simulink model "hybrid_pv_wind_feeder"  (R2024b)
settings: Solver=FixedStepDiscrete  StartTime=0.0  StopTime=1.0  FixedStep=P.Ts  RelTol=1e-3
model workspace (MAT data in the model file):
  P : object (value not decoded)
symbols that are objects in the model workspace (value not decoded): P
undefined symbols (not defined in the file): DiscIntNeverNeededParam
libraries: spsThreePhaseSeriesRLCBranchLib x28, spsSeriesRLCBranchLib x14, spsThreePhaseParallelRLCLoadLib x12, spsIGBTDiodeLib x8, slpidlib x7, spsThreePhaseBreakerLib x6, simulink x4, spsGroundLib x4, spsThreePhaseVIMeasurementLib x4, spsControlledCurrentSourceLib x3, spsDiodeLib x2, spsAlphaBetaZerotodq0Lib x2
(part 2 of 2)

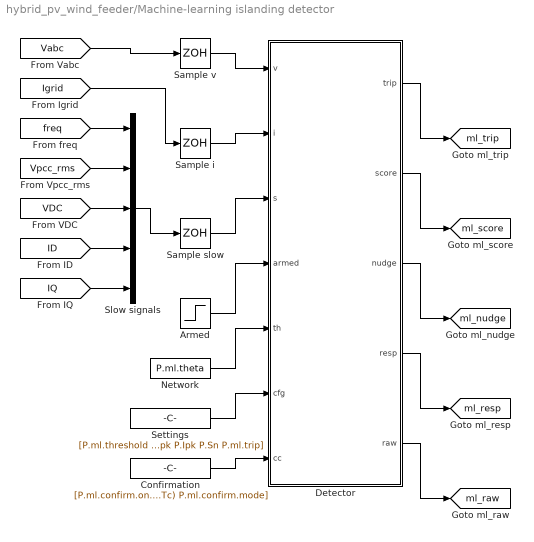
== system hybrid_pv_wind_feeder/Machine-learning islanding detector ==
  Armed : Step  Time=P.ml.tArm  SampleTime=P.Tc
  Confirmation : Constant  Value=[P.ml.confirm.on P.ml.confirm.amp round(P.ml.confirm.T/P.Tc) P.ml.confirm.thr P.ml.confirm.sign round(P.ml.confirm.hold/P.Tc) P.ml.confirm.mode]
  Detector : MATLAB Function  TreatAsAtomicUnit=on
  Network : Constant  Value=P.ml.theta
  Sample i : ZeroOrderHold  SampleTime=P.Tc
  Sample slow : ZeroOrderHold  SampleTime=P.Tc
  Sample v : ZeroOrderHold  SampleTime=P.Tc
  Settings : Constant  Value=[P.ml.threshold P.ml.debounce P.Vpk P.Ipk P.Sn P.ml.trip]
  Slow signals : Mux  Inputs=5
  tag scope: ml_nudge=global, ml_raw=global, ml_resp=global, ml_score=global, ml_trip=global
  wires:
  [freq] -> Slow signals/1
  [Vpcc_rms] -> Slow signals/2
  [VDC] -> Slow signals/3
  [ID] -> Slow signals/4
  [IQ] -> Slow signals/5
  [Vabc] -> Sample v/1
  [Igrid] -> Sample i/1
  Slow signals/1 -> Sample slow/1
  Sample v/1 -> Detector/1(v)
  Sample i/1 -> Detector/2(i)
  Sample slow/1 -> Detector/3(s)
  Armed/1 -> Detector/4(armed)
  Network/1 -> Detector/5(th)
  Settings/1 -> Detector/6(cfg)
  Confirmation/1 -> Detector/7(cc)
  Detector/1(trip) -> [ml_trip]
  Detector/2(score) -> [ml_score]
  Detector/3(nudge) -> [ml_nudge]
  Detector/4(resp) -> [ml_resp]
  Detector/5(raw) -> [ml_raw]

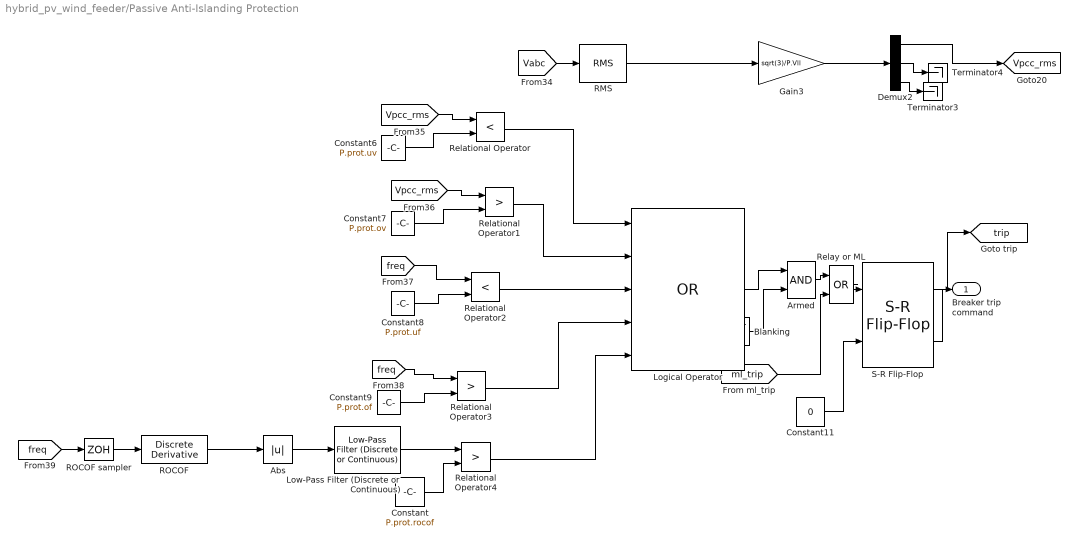
== system hybrid_pv_wind_feeder/Passive Anti-Islanding Protection ==
  Abs : Abs  SaturateOnIntegerOverflow=off
  Armed : Logic  AllPortsSameDT=off  OutDataTypeStr=boolean
  Blanking : Step  Time=P.prot.tArm  SampleTime=P.Ts
  Constant : Constant  Value=P.prot.rocof
  Constant11 : Constant  Value=0  VectorParams1D=off  OutDataTypeStr=boolean
  Constant6 : Constant  Value=P.prot.uv
  Constant7 : Constant  Value=P.prot.ov
  Constant8 : Constant  Value=P.prot.uf
  Constant9 : Constant  Value=P.prot.of
  Demux2 : Demux  Outputs=3
  Gain3 : Gain  Gain=sqrt(3)/P.Vll
  Logical Operator : Logic  Operator=OR  Inputs=5  AllPortsSameDT=off  OutDataTypeStr=boolean
  Low-Pass Filter (Discrete or Continuous) : eeGeneralControl/Low-Pass Filter (Discrete or Continuous)  K=1  T=1/(2*pi*10)  B=inf  A=-inf  init_option=Inherited from block input  x0=0  Ts=-1
  RMS : spsRMSLib/RMS  TrueRMS=on  Freq=P.fg  RMSInit=120  Ts=P.Ts
  ROCOF : simulink/Discrete/Discrete Derivative  gainval=1.0  ICPrevScaledInput=0.0  OutMin=[]  OutMax=[]  OutDataType=fixdt(1, 16)  OutScaling=2^-10  DoSatur=off
  ROCOF sampler : ZeroOrderHold  SampleTime=P.prot.Trocof
  Relational Operator : RelationalOperator  Operator=<  OutDataTypeStr=boolean  RndMeth=Simplest  InputSameDT=off
  Relational Operator1 : RelationalOperator  Operator=>  OutDataTypeStr=boolean  RndMeth=Simplest  InputSameDT=off
  Relational Operator2 : RelationalOperator  Operator=<  OutDataTypeStr=boolean  RndMeth=Simplest  InputSameDT=off
  Relational Operator3 : RelationalOperator  Operator=>  OutDataTypeStr=boolean  RndMeth=Simplest  InputSameDT=off
  Relational Operator4 : RelationalOperator  Operator=>  OutDataTypeStr=boolean  RndMeth=Simplest  InputSameDT=off
  Relay or ML : Logic  Operator=OR  AllPortsSameDT=off  OutDataTypeStr=boolean
  S-R Flip-Flop : simulink_extras/Flip Flops/S-R Flip-Flop  initial_condition=0
  Terminator3 : Terminator
  Terminator4 : Terminator
  "Breaker trip command " : Outport  VectorParamsAs1DForOutWhenUnconnected=off
  tag scope: Vpcc_rms=global, trip=global
  wires:
  RMS/1 -> Gain3/1
  Constant6/1 -> Relational Operator/2
  Constant7/1 -> Relational Operator1/2
  Abs/1 -> Low-Pass Filter (Discrete or Continuous)/1
  [Vpcc_rms] -> Relational Operator1/1
  Gain3/1 -> Demux2/1
  [Vabc] -> RMS/1
  [freq] -> Relational Operator3/1
  Low-Pass Filter (Discrete or Continuous)/1 -> Relational Operator4/1
  Constant11/1 -> S-R Flip-Flop/2
  Demux2/1 -> [Vpcc_rms]
  Constant8/1 -> Relational Operator2/2
  Constant/1 -> Relational Operator4/2
  Constant9/1 -> Relational Operator3/2
  [Vpcc_rms] -> Relational Operator/1
  Demux2/2 -> Terminator4/1
  Relational Operator1/1 -> Logical Operator/2
  Demux2/3 -> Terminator3/1
  Relational Operator3/1 -> Logical Operator/4
  Relational Operator/1 -> Logical Operator/1
  Relational Operator2/1 -> Logical Operator/3
  [freq] -> Relational Operator2/1
  Relational Operator4/1 -> Logical Operator/5
  [freq] -> ROCOF sampler/1
  ROCOF sampler/1 -> ROCOF/1
  ROCOF/1 -> Abs/1
  Logical Operator/1 -> Armed/1
  Blanking/1 -> Armed/2
  Armed/1 -> Relay or ML/1
  [ml_trip] -> Relay or ML/2
  Relay or ML/1 -> S-R Flip-Flop/1
  S-R Flip-Flop/2 -> "Breaker trip command "/1
  S-R Flip-Flop/1 -> [trip]

== system hybrid_pv_wind_feeder/Pwm Generator  ==
  1 : Inport
  Demux3 : Demux  Outputs=3
  Logical Operator1 : Logic  Operator=NOT  AllPortsSameDT=off  OutDataTypeStr=boolean
  Logical Operator2 : Logic  Operator=NOT  AllPortsSameDT=off  OutDataTypeStr=boolean
  Logical Operator3 : Logic  Operator=NOT  AllPortsSameDT=off  OutDataTypeStr=boolean
  Relational Operator : RelationalOperator  OutDataTypeStr=boolean  RndMeth=Simplest  InputSameDT=off
  Relational Operator1 : RelationalOperator  OutDataTypeStr=boolean  RndMeth=Simplest  InputSameDT=off
  Relational Operator2 : RelationalOperator  OutDataTypeStr=boolean  RndMeth=Simplest  InputSameDT=off
  Repeating Sequence : simulink/Sources/Repeating Sequence  rep_seq_t=[0 0.00005 0.0001]  rep_seq_y=[-1 1 -1]
  tag scope: PWM1=global, PWM2=global, PWM3=global, PWM4=global, PWM5=global, PWM6=global
  wires:
  Relational Operator/1 -> Logical Operator1/1, [PWM1]
  Demux3/2 -> Relational Operator1/1
  Demux3/1 -> Relational Operator/1
  Relational Operator1/1 -> [PWM3], Logical Operator2/1
  Repeating Sequence/1 -> Relational Operator1/2, Relational Operator/2, Relational Operator2/2
  Demux3/3 -> Relational Operator2/1
  1/1 -> Demux3/1
  Relational Operator2/1 -> [PWM5], Logical Operator3/1
  Logical Operator1/1 -> [PWM2]
  Logical Operator2/1 -> [PWM4]
  Logical Operator3/1 -> [PWM6]

== system hybrid_pv_wind_feeder/Second inverter control ==
  Armed : Step  Time=P.prot.tBlank  SampleTime=P.der2.Ts
  Current reference : MATLAB Function  TreatAsAtomicUnit=on
  Delay : UnitDelay  SampleTime=P.der2.Ts  HasFrameUpgradeWarning=on
  Enable : Step  Time=P.der2.tOn  After=P.der2.on  SampleTime=P.der2.Ts
  Sample : ZeroOrderHold  SampleTime=P.der2.Ts
  Sample freq : ZeroOrderHold  SampleTime=P.der2.Ts
  Settings : Constant  Value=[P.der2.P P.der2.Q P.der2.Kq P.der2.Qlim P.fg 1.5*(0.5*P.Vll*sqrt(2/3))^2 P.der2.Ts]
  Iabc ref : Outport
  wires:
  [Vder2] -> Sample/1
  Sample/1 -> Current reference/1(v)
  Enable/1 -> Current reference/3(en)
  Armed/1 -> Current reference/4(armed)
  Settings/1 -> Current reference/5(prm)
  Current reference/1(i) -> Delay/1
  Delay/1 -> Iabc ref/1
  [freq] -> Sample freq/1
  Sample freq/1 -> Current reference/2(f)

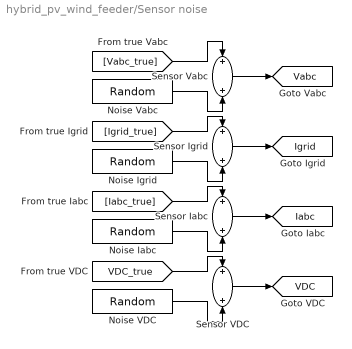
== system hybrid_pv_wind_feeder/Sensor noise ==
  Noise Iabc : RandomNumber  Variance=(P.noise.on*P.noise.i*P.Ipk)^2  Seed=10*P.noise.seed + [7 8 9]  SampleTime=P.Tc
  Noise Igrid : RandomNumber  Variance=(P.noise.on*P.noise.i*P.Ipk)^2  Seed=10*P.noise.seed + [4 5 6]  SampleTime=P.Tc
  Noise VDC : RandomNumber  Variance=(P.noise.on*P.noise.vdc*P.Vdc)^2  Seed=10*P.noise.seed + 10  SampleTime=P.Tc
  Noise Vabc : RandomNumber  Variance=(P.noise.on*P.noise.v*P.Vpk)^2  Seed=10*P.noise.seed + [1 2 3]  SampleTime=P.Tc
  Sensor Iabc : Sum
  Sensor Igrid : Sum
  Sensor VDC : Sum
  Sensor Vabc : Sum
  tag scope: Iabc=global, Igrid=global, VDC=global, Vabc=global
  wires:
  [Vabc_true] -> Sensor Vabc/1
  Noise Vabc/1 -> Sensor Vabc/2
  Sensor Vabc/1 -> [Vabc]
  [Igrid_true] -> Sensor Igrid/1
  Noise Igrid/1 -> Sensor Igrid/2
  Sensor Igrid/1 -> [Igrid]
  [Iabc_true] -> Sensor Iabc/1
  Noise Iabc/1 -> Sensor Iabc/2
  Sensor Iabc/1 -> [Iabc]
  [VDC_true] -> Sensor VDC/1
  Noise VDC/1 -> Sensor VDC/2
  Sensor VDC/1 -> [VDC]

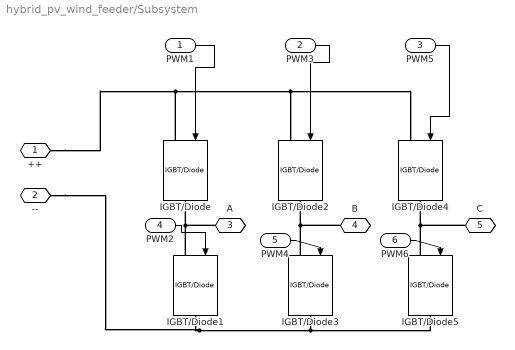
== system hybrid_pv_wind_feeder/Subsystem ==
  PWM1 : Inport
  PWM3 : Inport  Port=2
  PWM5 : Inport  Port=3
  PWM2 : Inport  Port=4
  PWM4 : Inport  Port=5
  PWM6 : Inport  Port=6
  IGBT/Diode{,1..5} (6 alike) : spsIGBTDiodeLib/IGBT//Diode  Ron=1e-3  Rs=1e5  Cs=inf  Measurements=off
  ++ : PMIOPort  Side=Left
  -- : PMIOPort  Port=2  Side=Left
  A : PMIOPort  Port=3  Side=Right
  B : PMIOPort  Port=4  Side=Right
  C : PMIOPort  Port=5  Side=Right
  wires:
  PWM1/1 -> IGBT/Diode/1
  PWM4/1 -> IGBT/Diode3/1
  PWM6/1 -> IGBT/Diode5/1
  PWM3/1 -> IGBT/Diode2/1
  PWM5/1 -> IGBT/Diode4/1
  PWM2/1 -> IGBT/Diode1/1
  connections:
  IGBT/Diode1/RConn1 -- --/RConn1 -- IGBT/Diode3/RConn1 -- IGBT/Diode5/RConn1
  IGBT/Diode3/LConn1 -- B/RConn1 -- IGBT/Diode2/RConn1
  IGBT/Diode1/LConn1 -- A/RConn1 -- IGBT/Diode/RConn1
  IGBT/Diode5/LConn1 -- C/RConn1 -- IGBT/Diode4/RConn1
  IGBT/Diode/LConn1 -- ++/RConn1 -- IGBT/Diode2/LConn1 -- IGBT/Diode4/LConn1

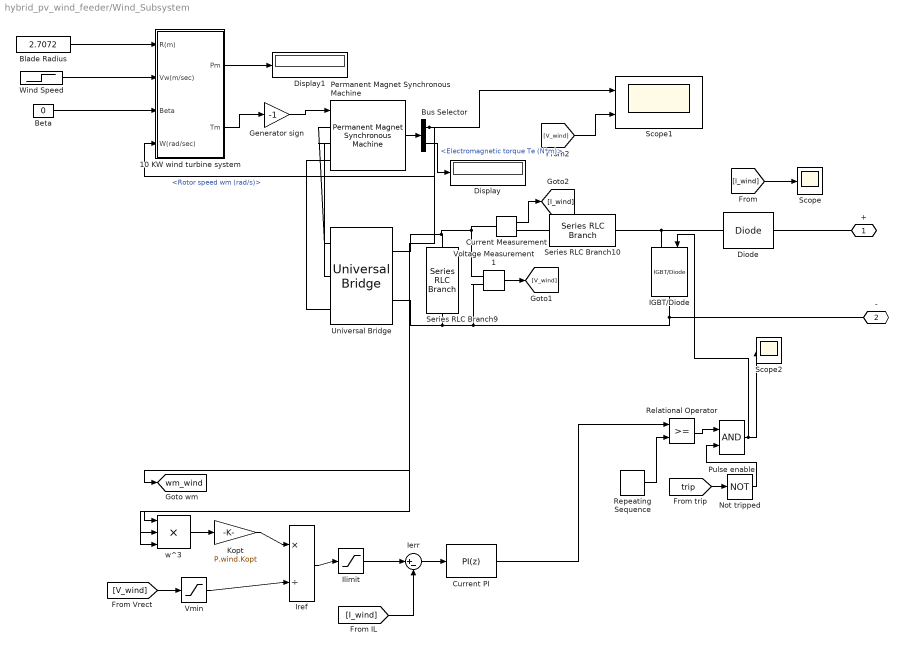
== system hybrid_pv_wind_feeder/Wind_Subsystem ==
  10 KW wind turbine system : Subsystem
  Beta : Constant  Value=0
  Blade Radius : Constant  Value=2.7072
  Bus Selector : BusSelector  OutputSignals=Rotor speed wm (rad/s),Electromagnetic torque Te (N*m)
  Current Measurement : spsCurrentMeasurementLib/Current Measurement  PhasorSimulation=off  OutputType=Complex  PSBequivalent=0
  Current PI : slpidlib/PID Controller  Controller=PI  Form=Parallel  TimeDomain=Discrete-time  UseExternalTs=off  SampleTime=-1  IntegratorMethod=Forward Euler  FilterMethod=Forward Euler  ControllerParametersSource=internal  P=P.wind.KpI  I=P.wind.KiI  UseKiTs=off  D=0  UseExternalDerivativeSource=off  N=100  UseFilter=on  TunerSelectOption=Transfer Function Based (PID Tuner App)  InitialConditionSource=internal  InitialConditionForIntegrator=P.wind.D0  InitialConditionForFilter=0  DifferentiatorICPrevScaledInput=0  ExternalReset=none  TrackingMode=off  Kt=1  LimitOutput=on  SatLimitsSource=internal  UpperSaturationLimit=0.92  LowerSaturationLimit=0  LinearizeAsGain=off  AntiWindupMode=clamping  Kb=1  LimitIntegrator=off  UpperIntegratorSaturationLimit=inf  LowerIntegratorSaturationLimit=-inf  POutMin=[]  POutMax=[]  IOutMin=[]  IOutMax=[]  DOutMin=[]  DOutMax=[]  NOutMin=[]  NOutMax=[]  SumOutMin=[]  SumOutMax=[]  SaturationOutMin=[]  SaturationOutMax=[]  PParamMin=[]  PParamMax=[]  IParamMin=[]  IParamMax=[]  DParamMin=[]  DParamMax=[]  NParamMin=[]  NParamMax=[]  KbParamMin=[]  KbParamMax=[]  KtParamMin=[]  KtParamMax=[]  KbOutMin=[]  KbOutMax=[]  KtOutMin=[]  KtOutMax=[]  IntegratorOutMin=[]  IntegratorOutMax=[]  FilterOutMin=[]  FilterOutMax=[]  SumI1OutMin=[]  SumI1OutMax=[]  SumI2OutMin=[]  SumI2OutMax=[]  SumI3OutMin=[]  SumI3OutMax=[]  SumI4OutMin=[]  SumI4OutMax=[]  SumDOutMin=[]  SumDOutMax=[]  DifferentiatorOutMin=[]  DifferentiatorOutMax=[]  FilterDiffOutCoefMin=[]  FilterDiffOutCoefMax=[]  ReciprocalOutMin=[]  ReciprocalOutMax=[]  SumDenOutMin=[]  SumDenOutMax=[]  SumNumOutMin=[]  SumNumOutMax=[]  DivideOutMin=[]  DivideOutMax=[]  UdiffTsProdOutMin=[]  UdiffTsProdOutMax=[]  NTsProdOutMin=[]  NTsProdOutMax=[]  UintegralTsProdOutMin=[]  UintegralTsProdOutMax=[]  UngainTsProdOutMin=[]  UngainTsProdOutMax=[]  ClampingZeroOutDataTypeStr=Inherit: Inherit via back propagation  ClampingZeroOutMin=[]  ClampingZeroOutMax=[]  FilterDenConstantOutDataTypeStr=Inherit: Inherit via back propagation  FilterDenConstantOutMin=[]  FilterDenConstantOutMax=[]  PCopyOutDataTypeStr=Inherit: Inherit via back propagation  PCopyOutMin=[]  PCopyOutMax=[]  NCopyOutDataTypeStr=Inherit: Inherit via back propagation  NCopyOutMin=[]  NCopyOutMax=[]  IntegratorContinuousStateAttributes=''  IntegratorStateMustResolveToSignalObject=off  IntegratorRTWStateStorageClass=Auto  FilterContinuousStateAttributes=''  FilterStateMustResolveToSignalObject=off  FilterRTWStateStorageClass=Auto  ParallelPVariant=InternalParameters  IdealPVariant=Disabled  IVariant=InternalParameters  DVariant=Disabled  IntegratorVariant=Discrete  SatVariant=Enabled  AWVariant=DiscClampingParallel  PCopyVariant=Disabled  TRVariant=Disabled  FdbkBlocksVariant=Forward  IdealPFdbkVariant=Disabled  SatFdbkVariant=Disabled  DerivativeFilterVariant=Disabled  NVariant=Disabled  NCopyVariant=Disabled_SignalSpec  FilterICVariant=Disabled  IntegratorICVariant=InternalICs  ExternalResetVariant=Disabled  TRSumVariant=Passthrough  SumFdbkVariant=Disabled  SumVariant=Sum_PI  TsampFilterVariant=InternalTs  TsampNgainVariant=Passthrough  TsampIntegralVariant=Disabled_SignalSpec  ExternalSaturationOutDataTypeStr=Inherit: Same as second input  DerivativeSourceVariant=Disabled  PreIntVariant=InternalPreInt
      settings: LibrarySourceBlock=simulink/Discrete/Discrete PID Controller
  Diode : spsDiodeLib/Diode  Ron=0.001  Lon=0  Vf=0.8  IC=0  UseSnubber=0  Rs=500  Cs=250e-9  Measurements=off
  Display : Display
  Display1 : Display
  Generator sign : Gain  Gain=-1
  IGBT/Diode : spsIGBTDiodeLib/IGBT//Diode  Ron=0.001  Rs=100  Cs=1e-6  Measurements=off
  Ierr : Sum  Inputs=|+-
  Ilimit : Saturate  UpperLimit=P.wind.Imax  LowerLimit=0
  Iref : Product  Inputs=*/
  Kopt : Gain  Gain=P.wind.Kopt
  Not tripped : Logic  Operator=NOT  AllPortsSameDT=off  OutDataTypeStr=boolean
  Permanent Magnet Synchronous Machine : spsPermanentMagnetSynchronousMachineLib/Permanent Magnet Synchronous Machine  NbPhases=3  FluxDistribution=Sinusoidal  RotorType=Round  MechanicalLoad=Torque Tm  PresetModel=No  ShowDetailedParameters=on  MeasurementBus=off  Resistance=0.05486  Inductance=P.wind.Ls  dqInductances=[P.wind.Ls P.wind.Ls]  La=0.000835  MachineConstant=Flux linkage established by magnets (V.s)  Flux=0.9  VoltageCst=652.9678  TorqueCst=5.4  Flat=120  Mechanical=[P.wind.J 0.008 P.wind.pp 0]  PolePairs=P.wind.pp  InitialConditions=[P.wind.wm0 0 0 0]  InitialConditions5ph=[0 0 0 0 0 0]  RefAngle=90 degrees behind phase A axis (modified Park)  IterativeDiscreteModel=Trapezoidal non iterative  TsBlock=-1  TsPowergui=0
  Pulse enable : Logic  AllPortsSameDT=off  OutDataTypeStr=boolean
  Relational Operator : RelationalOperator  OutDataTypeStr=boolean  RndMeth=Simplest  InputSameDT=off
  Repeating Sequence : simulink/Sources/Repeating Sequence  rep_seq_t="[0  0.0001]"  rep_seq_y=[0 1]
  Scope : Scope
  Scope1 : Scope  NumInputPorts=2
  Scope2 : Scope
  Series RLC Branch10 : spsSeriesRLCBranchLib/Series RLC Branch  LConnTagsString=__new0  RConnTagsString=__new0  BranchType=L  Resistance=2.3e-3  Inductance=10e-3  SetiL0=off  InitialCurrent=0  Capacitance=1e-6  Setx0=off  InitialVoltage=0  Measurements=None
  Series RLC Branch9 : spsSeriesRLCBranchLib/Series RLC Branch  LConnTagsString=__new0  RConnTagsString=__new0  BranchType=C  Resistance=1  Inductance=1e-3  SetiL0=off  InitialCurrent=0  Capacitance=2200e-6  Setx0=off  InitialVoltage=0  Measurements=None
  Universal Bridge : spsUniversalBridgeLib/Universal Bridge  Arms=3  SnubberResistance=5000  SnubberCapacitance=inf  Device=Diodes  Ron=0.001  Lon=0  ForwardVoltages="[  0  0  ]"  ForwardVoltage=0  GTOparameters=[ 10e-6 , 20e-6 ]  IGBTparameters=[ 1e-6 , 2e-6 ]  Measurements=None  Measurements_2=None  converterType=Rectifier
  Vmin : Saturate  UpperLimit=inf  LowerLimit=50
  Voltage Measurement1 : spsVoltageMeasurementLib/Voltage Measurement  PhasorSimulation=off  OutputType=Complex  PSBequivalent=0
  Wind Speed : Step  Time=P.wind.tStep  Before=P.wind.v0  After=P.wind.v1  SampleTime=0
  w^3 : Product  Inputs=3
  + : PMIOPort  Side=Right
  - : PMIOPort  Port=2  Side=Right
  tag scope: wm_wind=global
  wires:
  Bus Selector/1 -> Scope1/1, 10 KW wind turbine system/4(W(rad/sec)), w^3/1, w^3/2, w^3/3, [wm_wind]  "<Rotor speed wm (rad/s)>"
  [V_wind] -> Scope1/2
  Repeating Sequence/1 -> Relational Operator/2
  Permanent Magnet Synchronous Machine/1 -> Bus Selector/1
  Bus Selector/2 -> Display/1  "<Electromagnetic torque Te (N*m)>"
  Voltage Measurement1/1 -> [V_wind]
  Current Measurement/1 -> [I_wind]
  Beta/1 -> 10 KW wind turbine system/3(Beta)
  Blade Radius/1 -> 10 KW wind turbine system/1(R(m))
  10 KW wind turbine system/1(Pm) -> Display1/1
  Wind Speed/1 -> 10 KW wind turbine system/2(Vw(m/sec))
  [I_wind] -> Scope/1
  10 KW wind turbine system/2(Tm) -> Generator sign/1
  Generator sign/1 -> Permanent Magnet Synchronous Machine/1
  w^3/1 -> Kopt/1
  Kopt/1 -> Iref/1
  [V_wind] -> Vmin/1
  Vmin/1 -> Iref/2
  Iref/1 -> Ilimit/1
  Ilimit/1 -> Ierr/1
  [I_wind] -> Ierr/2
  Ierr/1 -> Current PI/1
  Current PI/1 -> Relational Operator/1
  [trip] -> Not tripped/1
  Relational Operator/1 -> Pulse enable/1
  Not tripped/1 -> Pulse enable/2
  Pulse enable/1 -> Scope2/1, IGBT/Diode/1
  connections:
  Series RLC Branch9/LConn1 -- Universal Bridge/RConn1 -- Voltage Measurement1/LConn1 -- Current Measurement/LConn1
  IGBT/Diode/RConn1 -- Voltage Measurement1/LConn2 -- Universal Bridge/RConn2 -- Series RLC Branch9/RConn1 -- -/RConn1
  Series RLC Branch10/RConn1 -- Diode/LConn1 -- IGBT/Diode/LConn1
  Diode/RConn1 -- +/RConn1
  Permanent Magnet Synchronous Machine/LConn2 -- Universal Bridge/LConn2
  Permanent Magnet Synchronous Machine/LConn1 -- Universal Bridge/LConn1
  Current Measurement/RConn1 -- Series RLC Branch10/LConn1
  Permanent Magnet Synchronous Machine/LConn3 -- Universal Bridge/LConn3

== system hybrid_pv_wind_feeder/Inverter Control Logic/Active frequency drift ==
  Add bias : Sum
  Add nudge : Sum
  Armed : Step  Time=P.prot.tBlank  After=P.afd.on  SampleTime=P.Tc
  Enable : Product
  Frequency error : Sum  Inputs=+-
  K : Gain  Gain=P.afd.K
  Limit : Saturate  UpperLimit=P.afd.lim  LowerLimit=-P.afd.lim
  bias : Constant  Value=P.afd.bias
  fg : Constant  Value=P.fg
  Iq ref : Outport
  wires:
  [freq] -> Frequency error/1
  fg/1 -> Frequency error/2
  Frequency error/1 -> K/1
  K/1 -> Add bias/1
  bias/1 -> Add bias/2
  Add bias/1 -> Limit/1
  Limit/1 -> Enable/1
  Armed/1 -> Enable/2
  Enable/1 -> Add nudge/1
  [ml_nudge] -> Add nudge/2
  Add nudge/1 -> Iq ref/1

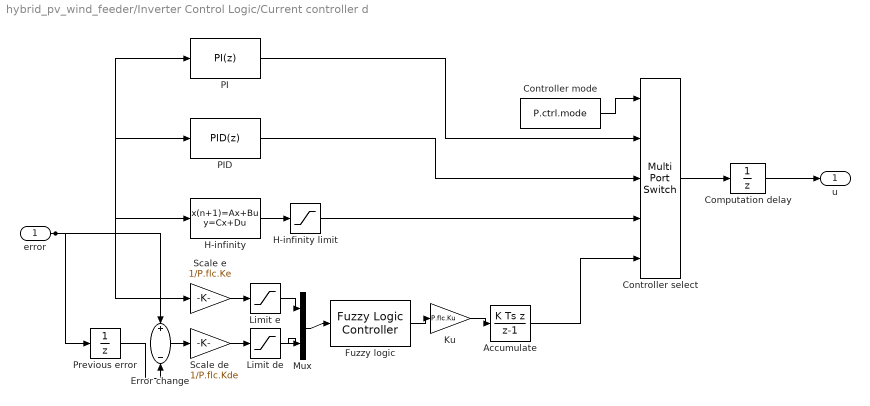
== system hybrid_pv_wind_feeder/Inverter Control Logic/Current controller d ==
  error : Inport
  Accumulate : DiscreteIntegrator  IntegratorMethod=Integration: Backward Euler  gainval=1/P.Tc  SampleTime=P.Tc  LimitOutput=on  UpperSaturationLimit=400  LowerSaturationLimit=-400  ICPrevOutput=DiscIntNeverNeededParam  ICPrevScaledInput=DiscIntNeverNeededParam
  Computation delay : UnitDelay  SampleTime=P.Tc  HasFrameUpgradeWarning=on
  Controller mode : Constant  Value=P.ctrl.mode
  Controller select : MultiPortSwitch  Inputs=4  SaturateOnIntegerOverflow=off  InputSameDT=off
  Error change : Sum  Inputs=+-
  Fuzzy logic : fuzblock/Fuzzy Logic  Controller  FIS=P.flc.fis  OutputSampleNumber=101  DataType=double  FuzzifiedInputs=off  RuleFiringStrengths=off  RuleOutputs=off  AggregatedOutputs=off  SimulateUsing=Code generation  OutOfRangeInputValueMessage=warning  NoRuleFiredMessage=warning  EmptyOutputFuzzySetMessage=warning
  H-infinity : DiscreteStateSpace  A=P.hinf.A  B=P.hinf.B  C=P.hinf.C  D=P.hinf.D  SampleTime=P.Tc
  H-infinity limit : Saturate  UpperLimit=400  LowerLimit=-400
  Ku : Gain  Gain=P.flc.Ku
  Limit de : Saturate  UpperLimit=1  LowerLimit=-1
  Limit e : Saturate  UpperLimit=1  LowerLimit=-1
  Mux : Mux  Inputs=2
  PI : slpidlib/PID Controller  Controller=PI  Form=Parallel  TimeDomain=Discrete-time  UseExternalTs=off  SampleTime=P.Tc  IntegratorMethod=Forward Euler  FilterMethod=Forward Euler  ControllerParametersSource=internal  P=P.ctrl.KpI  I=P.ctrl.KiI  UseKiTs=off  D=0  UseExternalDerivativeSource=off  N=100  UseFilter=on  TunerSelectOption=Transfer Function Based (PID Tuner App)  InitialConditionSource=internal  InitialConditionForIntegrator=0  InitialConditionForFilter=0  DifferentiatorICPrevScaledInput=0  ExternalReset=none  TrackingMode=off  Kt=1  LimitOutput=on  SatLimitsSource=internal  UpperSaturationLimit=400  LowerSaturationLimit=-400  LinearizeAsGain=on  AntiWindupMode=clamping  Kb=1  LimitIntegrator=off  UpperIntegratorSaturationLimit=inf  LowerIntegratorSaturationLimit=-inf  POutMin=[]  POutMax=[]  IOutMin=[]  IOutMax=[]  DOutMin=[]  DOutMax=[]  NOutMin=[]  NOutMax=[]  SumOutMin=[]  SumOutMax=[]  SaturationOutMin=[]  SaturationOutMax=[]  PParamMin=[]  PParamMax=[]  IParamMin=[]  IParamMax=[]  DParamMin=[]  DParamMax=[]  NParamMin=[]  NParamMax=[]  KbParamMin=[]  KbParamMax=[]  KtParamMin=[]  KtParamMax=[]  KbOutMin=[]  KbOutMax=[]  KtOutMin=[]  KtOutMax=[]  IntegratorOutMin=[]  IntegratorOutMax=[]  FilterOutMin=[]  FilterOutMax=[]  SumI1OutMin=[]  SumI1OutMax=[]  SumI2OutMin=[]  SumI2OutMax=[]  SumI3OutMin=[]  SumI3OutMax=[]  SumI4OutMin=[]  SumI4OutMax=[]  SumDOutMin=[]  SumDOutMax=[]  DifferentiatorOutMin=[]  DifferentiatorOutMax=[]  FilterDiffOutCoefMin=[]  FilterDiffOutCoefMax=[]  ReciprocalOutMin=[]  ReciprocalOutMax=[]  SumDenOutMin=[]  SumDenOutMax=[]  SumNumOutMin=[]  SumNumOutMax=[]  DivideOutMin=[]  DivideOutMax=[]  UdiffTsProdOutMin=[]  UdiffTsProdOutMax=[]  NTsProdOutMin=[]  NTsProdOutMax=[]  UintegralTsProdOutMin=[]  UintegralTsProdOutMax=[]  UngainTsProdOutMin=[]  UngainTsProdOutMax=[]  ClampingZeroOutDataTypeStr=Inherit: Inherit via back propagation  ClampingZeroOutMin=[]  ClampingZeroOutMax=[]  FilterDenConstantOutDataTypeStr=Inherit: Inherit via back propagation  FilterDenConstantOutMin=[]  FilterDenConstantOutMax=[]  PCopyOutDataTypeStr=Inherit: Inherit via back propagation  PCopyOutMin=[]  PCopyOutMax=[]  NCopyOutDataTypeStr=Inherit: Inherit via back propagation  NCopyOutMin=[]  NCopyOutMax=[]  IntegratorContinuousStateAttributes=''  IntegratorStateMustResolveToSignalObject=off  IntegratorRTWStateStorageClass=Auto  FilterContinuousStateAttributes=''  FilterStateMustResolveToSignalObject=off  FilterRTWStateStorageClass=Auto  ParallelPVariant=InternalParameters  IdealPVariant=Disabled  IVariant=InternalParameters  DVariant=Disabled  IntegratorVariant=Discrete  SatVariant=Enabled  AWVariant=DiscClampingParallel  PCopyVariant=Disabled  TRVariant=Disabled  FdbkBlocksVariant=Forward  IdealPFdbkVariant=Disabled  SatFdbkVariant=Disabled  DerivativeFilterVariant=Disabled  NVariant=Disabled  NCopyVariant=Disabled_SignalSpec  FilterICVariant=Disabled  IntegratorICVariant=InternalICs  ExternalResetVariant=Disabled  TRSumVariant=Passthrough  SumFdbkVariant=Disabled  SumVariant=Sum_PI  TsampFilterVariant=InternalTs  TsampNgainVariant=Passthrough  TsampIntegralVariant=Disabled_SignalSpec  ExternalSaturationOutDataTypeStr=Inherit: Same as second input  DerivativeSourceVariant=Disabled  PreIntVariant=InternalPreInt
  PID : slpidlib/PID Controller  Controller=PID  Form=Parallel  TimeDomain=Discrete-time  UseExternalTs=off  SampleTime=P.Tc  IntegratorMethod=Forward Euler  FilterMethod=Backward Euler  ControllerParametersSource=internal  P=P.pid.Kp  I=P.pid.Ki  UseKiTs=off  D=P.pid.Kd  UseExternalDerivativeSource=off  N=P.pid.N  UseFilter=on  TunerSelectOption=Transfer Function Based (PID Tuner App)  InitialConditionSource=internal  InitialConditionForIntegrator=0  InitialConditionForFilter=0  DifferentiatorICPrevScaledInput=0  ExternalReset=none  TrackingMode=off  Kt=1  LimitOutput=on  SatLimitsSource=internal  UpperSaturationLimit=400  LowerSaturationLimit=-400  LinearizeAsGain=off  AntiWindupMode=clamping  Kb=1  LimitIntegrator=off  UpperIntegratorSaturationLimit=inf  LowerIntegratorSaturationLimit=-inf  POutMin=[]  POutMax=[]  IOutMin=[]  IOutMax=[]  DOutMin=[]  DOutMax=[]  NOutMin=[]  NOutMax=[]  SumOutMin=[]  SumOutMax=[]  SaturationOutMin=[]  SaturationOutMax=[]  PParamMin=[]  PParamMax=[]  IParamMin=[]  IParamMax=[]  DParamMin=[]  DParamMax=[]  NParamMin=[]  NParamMax=[]  KbParamMin=[]  KbParamMax=[]  KtParamMin=[]  KtParamMax=[]  KbOutMin=[]  KbOutMax=[]  KtOutMin=[]  KtOutMax=[]  IntegratorOutMin=[]  IntegratorOutMax=[]  FilterOutMin=[]  FilterOutMax=[]  SumI1OutMin=[]  SumI1OutMax=[]  SumI2OutMin=[]  SumI2OutMax=[]  SumI3OutMin=[]  SumI3OutMax=[]  SumI4OutMin=[]  SumI4OutMax=[]  SumDOutMin=[]  SumDOutMax=[]  DifferentiatorOutMin=[]  DifferentiatorOutMax=[]  FilterDiffOutCoefMin=[]  FilterDiffOutCoefMax=[]  ReciprocalOutMin=[]  ReciprocalOutMax=[]  SumDenOutMin=[]  SumDenOutMax=[]  SumNumOutMin=[]  SumNumOutMax=[]  DivideOutMin=[]  DivideOutMax=[]  UdiffTsProdOutMin=[]  UdiffTsProdOutMax=[]  NTsProdOutMin=[]  NTsProdOutMax=[]  UintegralTsProdOutMin=[]  UintegralTsProdOutMax=[]  UngainTsProdOutMin=[]  UngainTsProdOutMax=[]  ClampingZeroOutDataTypeStr=Inherit: Inherit via back propagation  ClampingZeroOutMin=[]  ClampingZeroOutMax=[]  FilterDenConstantOutDataTypeStr=Inherit: Inherit via back propagation  FilterDenConstantOutMin=[]  FilterDenConstantOutMax=[]  PCopyOutDataTypeStr=Inherit: Inherit via back propagation  PCopyOutMin=[]  PCopyOutMax=[]  NCopyOutDataTypeStr=Inherit: Inherit via back propagation  NCopyOutMin=[]  NCopyOutMax=[]  IntegratorContinuousStateAttributes=''  IntegratorStateMustResolveToSignalObject=off  IntegratorRTWStateStorageClass=Auto  FilterContinuousStateAttributes=''  FilterStateMustResolveToSignalObject=off  FilterRTWStateStorageClass=Auto  ParallelPVariant=InternalParameters  IdealPVariant=Disabled  IVariant=InternalParameters  DVariant=InternalParameters  IntegratorVariant=Discrete  SatVariant=Enabled  AWVariant=DiscClampingParallel  PCopyVariant=Disabled  TRVariant=Disabled  FdbkBlocksVariant=Forward  IdealPFdbkVariant=Disabled  SatFdbkVariant=Disabled  DerivativeFilterVariant=BackwardEulerFilter  NVariant=InternalParameters  NCopyVariant=InternalParameters  FilterICVariant=InternalICsFilter  IntegratorICVariant=InternalICs  ExternalResetVariant=Disabled  TRSumVariant=Passthrough  SumFdbkVariant=Disabled  SumVariant=Sum_PID  TsampFilterVariant=InternalTs  TsampNgainVariant=Passthrough  TsampIntegralVariant=Disabled_SignalSpec  ExternalSaturationOutDataTypeStr=Inherit: Same as second input  DerivativeSourceVariant=ErrorSignal  PreIntVariant=InternalPreInt
      settings: LibrarySourceBlock=simulink/Discrete/Discrete PID Controller
  Previous error : UnitDelay  SampleTime=P.Tc  HasFrameUpgradeWarning=on
  Scale de : Gain  Gain=1/P.flc.Kde
  Scale e : Gain  Gain=1/P.flc.Ke
  u : Outport
  wires:
  error/1 -> PI/1, PID/1, H-infinity/1, Previous error/1, Error change/1, Scale e/1
  Previous error/1 -> Error change/2
  Error change/1 -> Scale de/1
  Scale e/1 -> Limit e/1
  Scale de/1 -> Limit de/1
  Limit e/1 -> Mux/1
  Limit de/1 -> Mux/2
  Mux/1 -> Fuzzy logic/1
  Fuzzy logic/1 -> Ku/1
  Ku/1 -> Accumulate/1
  H-infinity/1 -> H-infinity limit/1
  Controller mode/1 -> Controller select/1
  PI/1 -> Controller select/2
  PID/1 -> Controller select/3
  H-infinity limit/1 -> Controller select/4
  Accumulate/1 -> Controller select/5
  Controller select/1 -> Computation delay/1
  Computation delay/1 -> u/1

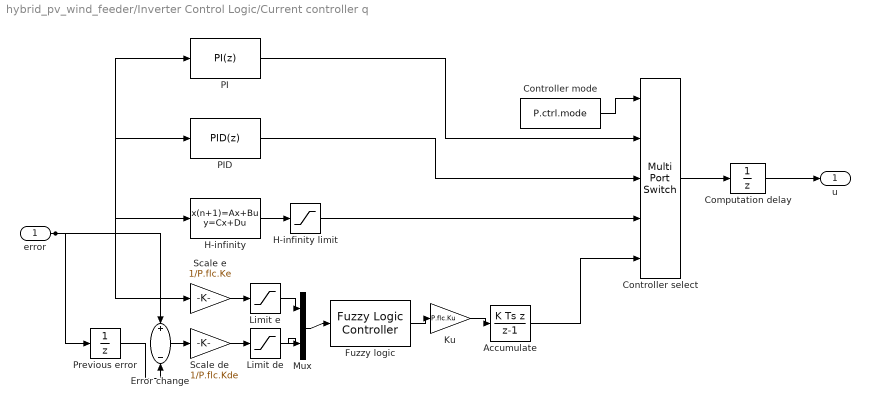
== system hybrid_pv_wind_feeder/Inverter Control Logic/Current controller q ==
  error : Inport
  Accumulate : DiscreteIntegrator  IntegratorMethod=Integration: Backward Euler  gainval=1/P.Tc  SampleTime=P.Tc  LimitOutput=on  UpperSaturationLimit=400  LowerSaturationLimit=-400  ICPrevOutput=DiscIntNeverNeededParam  ICPrevScaledInput=DiscIntNeverNeededParam
  Computation delay : UnitDelay  SampleTime=P.Tc  HasFrameUpgradeWarning=on
  Controller mode : Constant  Value=P.ctrl.mode
  Controller select : MultiPortSwitch  Inputs=4  SaturateOnIntegerOverflow=off  InputSameDT=off
  Error change : Sum  Inputs=+-
  Fuzzy logic : fuzblock/Fuzzy Logic  Controller  FIS=P.flc.fis  OutputSampleNumber=101  DataType=double  FuzzifiedInputs=off  RuleFiringStrengths=off  RuleOutputs=off  AggregatedOutputs=off  SimulateUsing=Code generation  OutOfRangeInputValueMessage=warning  NoRuleFiredMessage=warning  EmptyOutputFuzzySetMessage=warning
  H-infinity : DiscreteStateSpace  A=P.hinf.A  B=P.hinf.B  C=P.hinf.C  D=P.hinf.D  SampleTime=P.Tc
  H-infinity limit : Saturate  UpperLimit=400  LowerLimit=-400
  Ku : Gain  Gain=P.flc.Ku
  Limit de : Saturate  UpperLimit=1  LowerLimit=-1
  Limit e : Saturate  UpperLimit=1  LowerLimit=-1
  Mux : Mux  Inputs=2
  PI : slpidlib/PID Controller  Controller=PI  Form=Parallel  TimeDomain=Discrete-time  UseExternalTs=off  SampleTime=P.Tc  IntegratorMethod=Forward Euler  FilterMethod=Forward Euler  ControllerParametersSource=internal  P=P.ctrl.KpI  I=P.ctrl.KiI  UseKiTs=off  D=0  UseExternalDerivativeSource=off  N=100  UseFilter=on  TunerSelectOption=Transfer Function Based (PID Tuner App)  InitialConditionSource=internal  InitialConditionForIntegrator=0  InitialConditionForFilter=0  DifferentiatorICPrevScaledInput=0  ExternalReset=none  TrackingMode=off  Kt=1  LimitOutput=off  SatLimitsSource=internal  UpperSaturationLimit=inf  LowerSaturationLimit=-inf  LinearizeAsGain=on  AntiWindupMode=none  Kb=1  LimitIntegrator=off  UpperIntegratorSaturationLimit=inf  LowerIntegratorSaturationLimit=-inf  POutMin=[]  POutMax=[]  IOutMin=[]  IOutMax=[]  DOutMin=[]  DOutMax=[]  NOutMin=[]  NOutMax=[]  SumOutMin=[]  SumOutMax=[]  SaturationOutMin=[]  SaturationOutMax=[]  PParamMin=[]  PParamMax=[]  IParamMin=[]  IParamMax=[]  DParamMin=[]  DParamMax=[]  NParamMin=[]  NParamMax=[]  KbParamMin=[]  KbParamMax=[]  KtParamMin=[]  KtParamMax=[]  KbOutMin=[]  KbOutMax=[]  KtOutMin=[]  KtOutMax=[]  IntegratorOutMin=[]  IntegratorOutMax=[]  FilterOutMin=[]  FilterOutMax=[]  SumI1OutMin=[]  SumI1OutMax=[]  SumI2OutMin=[]  SumI2OutMax=[]  SumI3OutMin=[]  SumI3OutMax=[]  SumI4OutMin=[]  SumI4OutMax=[]  SumDOutMin=[]  SumDOutMax=[]  DifferentiatorOutMin=[]  DifferentiatorOutMax=[]  FilterDiffOutCoefMin=[]  FilterDiffOutCoefMax=[]  ReciprocalOutMin=[]  ReciprocalOutMax=[]  SumDenOutMin=[]  SumDenOutMax=[]  SumNumOutMin=[]  SumNumOutMax=[]  DivideOutMin=[]  DivideOutMax=[]  UdiffTsProdOutMin=[]  UdiffTsProdOutMax=[]  NTsProdOutMin=[]  NTsProdOutMax=[]  UintegralTsProdOutMin=[]  UintegralTsProdOutMax=[]  UngainTsProdOutMin=[]  UngainTsProdOutMax=[]  ClampingZeroOutDataTypeStr=Inherit: Inherit via back propagation  ClampingZeroOutMin=[]  ClampingZeroOutMax=[]  FilterDenConstantOutDataTypeStr=Inherit: Inherit via back propagation  FilterDenConstantOutMin=[]  FilterDenConstantOutMax=[]  PCopyOutDataTypeStr=Inherit: Inherit via back propagation  PCopyOutMin=[]  PCopyOutMax=[]  NCopyOutDataTypeStr=Inherit: Inherit via back propagation  NCopyOutMin=[]  NCopyOutMax=[]  IntegratorContinuousStateAttributes=''  IntegratorStateMustResolveToSignalObject=off  IntegratorRTWStateStorageClass=Auto  FilterContinuousStateAttributes=''  FilterStateMustResolveToSignalObject=off  FilterRTWStateStorageClass=Auto  ParallelPVariant=InternalParameters  IdealPVariant=Disabled  IVariant=InternalParameters  DVariant=Disabled  IntegratorVariant=Discrete  SatVariant=Disabled  AWVariant=Passthrough  PCopyVariant=Disabled  TRVariant=Disabled  FdbkBlocksVariant=Forward  IdealPFdbkVariant=Disabled  SatFdbkVariant=Disabled  DerivativeFilterVariant=Disabled  NVariant=Disabled  NCopyVariant=Disabled_SignalSpec  FilterICVariant=Disabled  IntegratorICVariant=InternalICs  ExternalResetVariant=Disabled  TRSumVariant=Passthrough  SumFdbkVariant=Disabled  SumVariant=Sum_PI  TsampFilterVariant=InternalTs  TsampNgainVariant=Passthrough  TsampIntegralVariant=Disabled_SignalSpec  ExternalSaturationOutDataTypeStr=Inherit: Same as second input  DerivativeSourceVariant=Disabled  PreIntVariant=InternalPreInt
  PID : slpidlib/PID Controller  Controller=PID  Form=Parallel  TimeDomain=Discrete-time  UseExternalTs=off  SampleTime=P.Tc  IntegratorMethod=Forward Euler  FilterMethod=Backward Euler  ControllerParametersSource=internal  P=P.pid.Kp  I=P.pid.Ki  UseKiTs=off  D=P.pid.Kd  UseExternalDerivativeSource=off  N=P.pid.N  UseFilter=on  TunerSelectOption=Transfer Function Based (PID Tuner App)  InitialConditionSource=internal  InitialConditionForIntegrator=0  InitialConditionForFilter=0  DifferentiatorICPrevScaledInput=0  ExternalReset=none  TrackingMode=off  Kt=1  LimitOutput=on  SatLimitsSource=internal  UpperSaturationLimit=400  LowerSaturationLimit=-400  LinearizeAsGain=off  AntiWindupMode=clamping  Kb=1  LimitIntegrator=off  UpperIntegratorSaturationLimit=inf  LowerIntegratorSaturationLimit=-inf  POutMin=[]  POutMax=[]  IOutMin=[]  IOutMax=[]  DOutMin=[]  DOutMax=[]  NOutMin=[]  NOutMax=[]  SumOutMin=[]  SumOutMax=[]  SaturationOutMin=[]  SaturationOutMax=[]  PParamMin=[]  PParamMax=[]  IParamMin=[]  IParamMax=[]  DParamMin=[]  DParamMax=[]  NParamMin=[]  NParamMax=[]  KbParamMin=[]  KbParamMax=[]  KtParamMin=[]  KtParamMax=[]  KbOutMin=[]  KbOutMax=[]  KtOutMin=[]  KtOutMax=[]  IntegratorOutMin=[]  IntegratorOutMax=[]  FilterOutMin=[]  FilterOutMax=[]  SumI1OutMin=[]  SumI1OutMax=[]  SumI2OutMin=[]  SumI2OutMax=[]  SumI3OutMin=[]  SumI3OutMax=[]  SumI4OutMin=[]  SumI4OutMax=[]  SumDOutMin=[]  SumDOutMax=[]  DifferentiatorOutMin=[]  DifferentiatorOutMax=[]  FilterDiffOutCoefMin=[]  FilterDiffOutCoefMax=[]  ReciprocalOutMin=[]  ReciprocalOutMax=[]  SumDenOutMin=[]  SumDenOutMax=[]  SumNumOutMin=[]  SumNumOutMax=[]  DivideOutMin=[]  DivideOutMax=[]  UdiffTsProdOutMin=[]  UdiffTsProdOutMax=[]  NTsProdOutMin=[]  NTsProdOutMax=[]  UintegralTsProdOutMin=[]  UintegralTsProdOutMax=[]  UngainTsProdOutMin=[]  UngainTsProdOutMax=[]  ClampingZeroOutDataTypeStr=Inherit: Inherit via back propagation  ClampingZeroOutMin=[]  ClampingZeroOutMax=[]  FilterDenConstantOutDataTypeStr=Inherit: Inherit via back propagation  FilterDenConstantOutMin=[]  FilterDenConstantOutMax=[]  PCopyOutDataTypeStr=Inherit: Inherit via back propagation  PCopyOutMin=[]  PCopyOutMax=[]  NCopyOutDataTypeStr=Inherit: Inherit via back propagation  NCopyOutMin=[]  NCopyOutMax=[]  IntegratorContinuousStateAttributes=''  IntegratorStateMustResolveToSignalObject=off  IntegratorRTWStateStorageClass=Auto  FilterContinuousStateAttributes=''  FilterStateMustResolveToSignalObject=off  FilterRTWStateStorageClass=Auto  ParallelPVariant=InternalParameters  IdealPVariant=Disabled  IVariant=InternalParameters  DVariant=InternalParameters  IntegratorVariant=Discrete  SatVariant=Enabled  AWVariant=DiscClampingParallel  PCopyVariant=Disabled  TRVariant=Disabled  FdbkBlocksVariant=Forward  IdealPFdbkVariant=Disabled  SatFdbkVariant=Disabled  DerivativeFilterVariant=BackwardEulerFilter  NVariant=InternalParameters  NCopyVariant=InternalParameters  FilterICVariant=InternalICsFilter  IntegratorICVariant=InternalICs  ExternalResetVariant=Disabled  TRSumVariant=Passthrough  SumFdbkVariant=Disabled  SumVariant=Sum_PID  TsampFilterVariant=InternalTs  TsampNgainVariant=Passthrough  TsampIntegralVariant=Disabled_SignalSpec  ExternalSaturationOutDataTypeStr=Inherit: Same as second input  DerivativeSourceVariant=ErrorSignal  PreIntVariant=InternalPreInt
      settings: LibrarySourceBlock=simulink/Discrete/Discrete PID Controller
  Previous error : UnitDelay  SampleTime=P.Tc  HasFrameUpgradeWarning=on
  Scale de : Gain  Gain=1/P.flc.Kde
  Scale e : Gain  Gain=1/P.flc.Ke
  u : Outport
  wires:
  error/1 -> PI/1, PID/1, H-infinity/1, Previous error/1, Error change/1, Scale e/1
  Previous error/1 -> Error change/2
  Error change/1 -> Scale de/1
  Scale e/1 -> Limit e/1
  Scale de/1 -> Limit de/1
  Limit e/1 -> Mux/1
  Limit de/1 -> Mux/2
  Mux/1 -> Fuzzy logic/1
  Fuzzy logic/1 -> Ku/1
  Ku/1 -> Accumulate/1
  H-infinity/1 -> H-infinity limit/1
  Controller mode/1 -> Controller select/1
  PI/1 -> Controller select/2
  PID/1 -> Controller select/3
  H-infinity limit/1 -> Controller select/4
  Accumulate/1 -> Controller select/5
  Controller select/1 -> Computation delay/1
  Computation delay/1 -> u/1

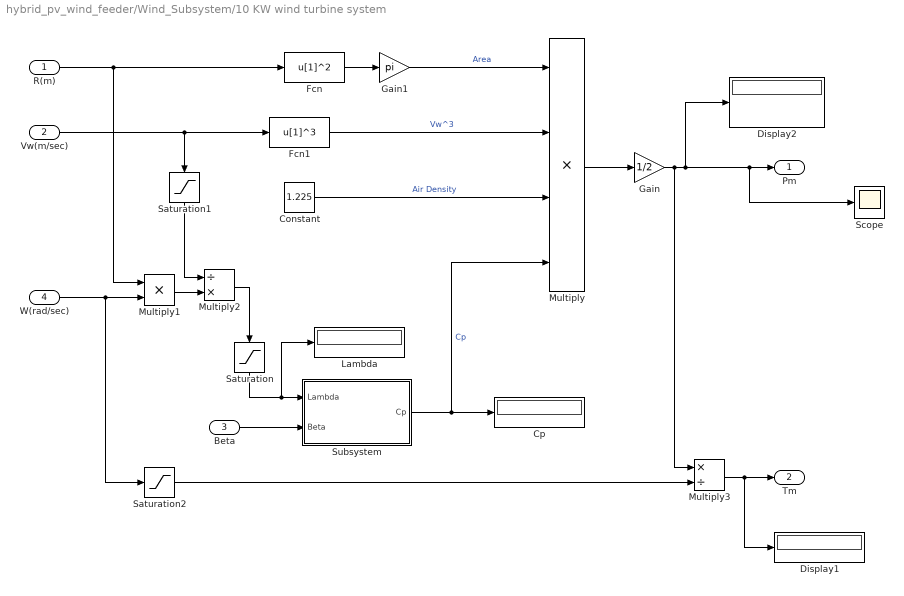
== system hybrid_pv_wind_feeder/Wind_Subsystem/10 KW wind turbine system ==
  R(m) : Inport
  Vw(m/sec) : Inport  Port=2
  Beta : Inport  Port=3
  W(rad/sec) : Inport  Port=4
  Constant : Constant  Value=1.225
  Cp : Display
  Display1 : Display
  Display2 : Display
  Fcn : Fcn  Expr=u[1]^2
  Fcn1 : Fcn  Expr=u[1]^3
  Gain : Gain  Gain=1/2
  Gain1 : Gain  Gain=pi
  Lambda : Display
  Multiply : Product  Inputs=4
  Multiply1 : Product
  Multiply2 : Product  Inputs=/*
  Multiply3 : Product  Inputs=*/
  Saturation : Saturate  UpperLimit=inf  LowerLimit=1e-6
  Saturation1 : Saturate  UpperLimit=inf  LowerLimit=1e-6
  Saturation2 : Saturate  UpperLimit=inf  LowerLimit=1e-6
  Scope : Scope
  Subsystem : Subsystem
  Pm : Outport  VectorParamsAs1DForOutWhenUnconnected=off
  Tm : Outport  Port=2  VectorParamsAs1DForOutWhenUnconnected=off
  wires:
  Gain/1 -> Multiply3/1, Display2/1, Scope/1, Pm/1
  Multiply/1 -> Gain/1
  Gain1/1 -> Multiply/1  "Area"
  Fcn1/1 -> Multiply/2  "Vw^3"
  Constant/1 -> Multiply/3  "Air Density"
  Subsystem/1(Cp) -> Cp/1, Multiply/4  "Cp"
  Fcn/1 -> Gain1/1
  R(m)/1 -> Multiply1/1, Fcn/1
  Vw(m/sec)/1 -> Fcn1/1, Saturation1/1
  Beta/1 -> Subsystem/2(Beta)
  W(rad/sec)/1 -> Saturation2/1, Multiply1/2
  Multiply1/1 -> Multiply2/2
  Multiply2/1 -> Saturation/1
  Saturation1/1 -> Multiply2/1
  Saturation2/1 -> Multiply3/2
  Multiply3/1 -> Display1/1, Tm/1
  Saturation/1 -> Lambda/1, Subsystem/1(Lambda)

== system hybrid_pv_wind_feeder/Wind_Subsystem/10 KW wind turbine system/Subsystem ==
  Lambda : Inport
  Beta : Inport  Port=2
  Eqn 2 : Fcn  Expr=0.5*(116*u[1]-0.4*u[2]-5)*exp(-21*u[1])
  Eqn3 : Fcn  Expr=1/(u[1]+0.08*u[2])-0.035/(1+u[2]^3)
  Mux : Mux  Inputs=2
  Mux1 : Mux  Inputs=2
  Cp : Outport  VectorParamsAs1DForOutWhenUnconnected=off
  wires:
  Eqn 2/1 -> Cp/1
  Mux/1 -> Eqn 2/1
  Lambda/1 -> Mux1/1  "u[1]"
  Eqn3/1 -> Mux/1  "u[1]"
  Beta/1 -> Mux1/2, Mux/2  "u[2]"
  Mux1/1 -> Eqn3/1

== matlab function hybrid_pv_wind_feeder/Second inverter control/Current reference ==
  data: v input; i output; f input; en input; armed input; prm input
function i = DER2(v, f, en, armed, prm)
% Constant-power current references from the fundamental of the terminal voltage.
persistent x1 x2
if isempty(x1), x1 = zeros(3, 1); x2 = zeros(3, 1); end
w = 2*pi*min(max(f, 40), 60); Ts = prm(7); k = sqrt(2);
x1n = x1 + Ts*w*(k*(v(:) - x1) - x2);   % SOGI: x1 in phase with v, x2 lagging 90 degrees
x2 = x2 + Ts*w*x1;
x1 = x1n;
Pd = prm(1);
Q = prm(2) + armed*min(max(prm(3)*(f - prm(5)), -prm(4)), prm(4));
v90 = [x1(2) - x1(3); x1(3) - x1(1); x1(1) - x1(2)]/sqrt(3);
s = max(x1(1)^2 + x1(2)^2 + x1(3)^2, prm(6));
i = en*(Pd*x1 - Q*v90)/s;

== matlab function hybrid_pv_wind_feeder/DC-DC Boost Converter with MPPT/MPPT ==
  data: V input; D output; I input
function D = MPPT(V,I)
% Perturb and observe on the boost duty cycle.
% A higher duty lowers the PV voltage, since Vpv = Vdc*(1-D).
Dmin = 0.5875; Dmax = 0.7125; D0 = 0.6375; dD = 0.003;
persistent Vold Pold Dold;
if isempty(Vold)
    Vold = V; Pold = V*I; Dold = D0;
end
P = V*I; dV = V - Vold; dP = P - Pold;
D = Dold;
if dP ~= 0
    if (dP > 0) == (dV > 0)
        D = Dold - dD;   % raise the voltage
    else
        D = Dold + dD;   % lower the voltage
    end
end
D = min(max(D, Dmin), Dmax);
Dold = D; Vold = V; Pold = P;

== matlab function hybrid_pv_wind_feeder/Machine-learning islanding detector/Detector ==
  data: v input; trip output; i input; s input; armed input; th input; cfg input; cc input; score output; nudge output; resp output; raw output
function [trip, score, nudge, resp, raw] = ML(v, i, s, armed, th, cfg, cc)
% Sliding-window islanding detector: features (ML_FEATURES) and a neural network.
% s = [frequency; RMS voltage; DC-link voltage; Id; Iq]; cfg = [threshold debounce Vpk Ipk Sn trip].
% cc = [on amp samples thr sign hold mode] (P.ml.confirm): with on > 0 an alarm starts a
% q-current nudge of amp for the given samples and trips only if the PCC voltage angle
% then moves by more than thr (resp: drift of the two cycles before removed; raw: not).
NB = 400; NW = 200; MB = 40; MW = 20; DEC = 10; EVERY = 50; NF = 22; H1 = 20; H2 = 10; NC = 200;
persistent bv bi bs k run sc tr conf hld P0 r rs rw
if isempty(k)
    bv = zeros(NB + NW + 1, 3); bi = zeros(NB + NW + 1, 3); bs = zeros(MB + MW + 1, 5);
    k = 0; run = 0; sc = 0; tr = 0; conf = 0; hld = 0; P0 = complex(0, 0); r = 0; rs = 0; rw = 0;
end
bv = [bv(2:end,:); v(:).'];  bi = [bi(2:end,:); i(:).'];
if mod(k, DEC) == 0, bs = [bs(2:end,:); s(:).']; end
if armed > 0 && mod(k, EVERY) == 0 && k >= NB + NW
    x = ml_features(bv, bi, bs(:,1), bs(:,3), bs(:,4), bs(:,5), MW, NW, cfg(3), cfg(4), cfg(5), 1000, 10000);
    z = (x(:) - th(1:NF))./th(NF+1:2*NF); o = 2*NF;
    W1 = reshape(th(o+1:o+H1*NF), H1, NF); o = o + H1*NF; b1 = th(o+1:o+H1); o = o + H1;
    W2 = reshape(th(o+1:o+H2*H1), H2, H1); o = o + H2*H1; b2 = th(o+1:o+H2); o = o + H2;
    W3 = reshape(th(o+1:o+2*H2), 2, H2); o = o + 2*H2; b3 = th(o+1:o+2);
    a = W3*max(W2*max(W1*z + b1, 0) + b2, 0) + b3;
    sc = 1/(1 + exp(a(1) - a(2)));
    if sc > cfg(1) && conf == 0 && hld == 0, run = run + 1; else, run = 0; end
    if run >= cfg(2) && cfg(6) > 0 && tr == 0
        run = 0;
        if cc(1) > 0
            conf = 1; P0 = cycle_phasor(bv, k, 0, NC, cfg(3));
            r = angle(P0*conj(cycle_phasor(bv, k, NC, NC, cfg(3))));
        else
            tr = 1;
        end
    end
end
if conf > cc(3)
    P1 = cycle_phasor(bv, k, 0, NC, cfg(3));
    rw = angle(P1*conj(P0)); rs = angle(P1*conj(P0)*exp(-1i*r*cc(3)/NC));
    d = rs; if cc(7) > 1, d = rw; end
    if cc(5) ~= 0, d = cc(5)*d; else, d = abs(d); end
    if d > cc(4), tr = 1; else, hld = cc(6); end
    conf = 0;
elseif conf > 0
    conf = conf + 1;
elseif hld > 0
    hld = hld - 1;
end
k = k + 1;
trip = tr; score = sc; nudge = cc(2)*(conf > 0); resp = rs; raw = rw;

function P = cycle_phasor(bv, k, lag, NC, Vpk)
% Positive-sequence voltage phasor (pu) of the cycle ending LAG samples ago, at 50 Hz.
j = (size(bv, 1) - lag - NC + (1:NC)).';      % rows; the newest row is sample k
m = (k - lag - NC + (1:NC)).';
a = exp(1i*2*pi/3);
x = (bv(j,1) + a*bv(j,2) + a*a*bv(j,3))*(2/(3*Vpk));
P = mean(x.*exp(-1i*2*pi*m/NC));
